simulink model "GD32__HOST"  (R2024a)
settings: Solver=FixedStepDiscrete  StartTime=0.0  StopTime=inf  FixedStep=0.1  RelTol=1e-3
libraries: instrumentseriallib x3
settings Model: Creator=33595  LastModifiedBy=ZJH
settings SolverCC: AlgebraicLoopSolver=TrustRegion
settings DataIOCC: ReturnWorkspaceOutputs=off
settings DebuggingCC: UnconnectedInputMsg=warning  UnconnectedOutputMsg=warning  UnconnectedLineMsg=warning
settings ModelReferenceCC: EnableRefExpFcnMdlSchedulingChecks=on
settings SFSimCC: CustomCodeUndefinedFunction=UseInterfaceOnly
settings RTWCC: GPUComputeCapability=3.5  DLArmComputeVersion=19.05

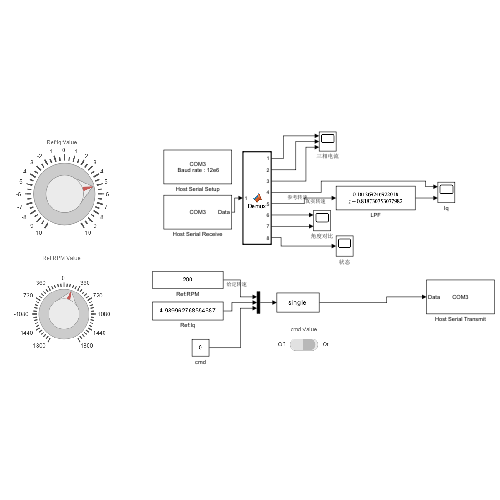
[thumbnail: Simulink's stored preview of the top-level diagram]
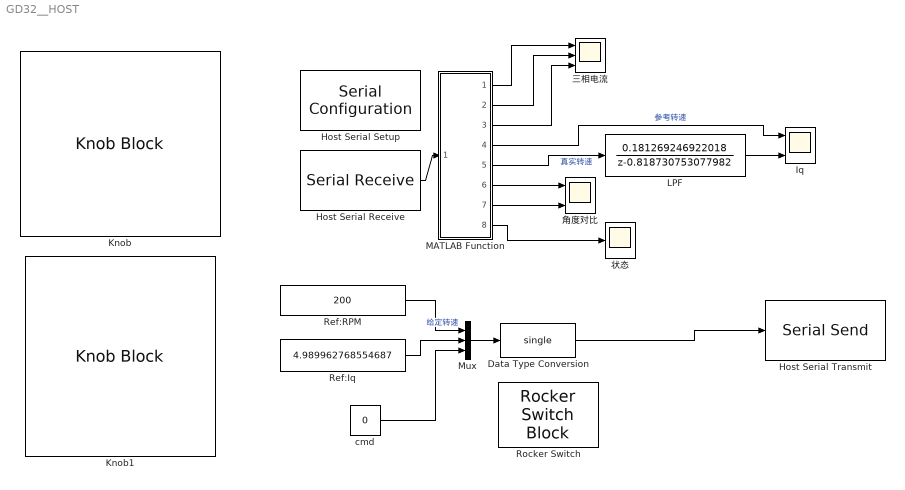
== system GD32__HOST ==
  Data Type Conversion : DataTypeConversion  OutDataTypeStr=single  SaturateOnIntegerOverflow=off  RndMeth=Floor
  Host Serial Receive : instrumentseriallib/Serial Receive  PortSel=COM3  Port=COM3  ComPort=COM3  DataType=single  SaveDataType=uint8  ToggleHeader=off  Header='PMSM'  ToggleDataSize=on  DataSize=[1000 8]  ToggleTerminator=off  Terminator=Custom terminator  CustomTerminator='ATJC'  InputFormat=Row major  EnableBlockingMode=on  ActionDataUnavailable=Output custom value  ActionWhenDataUnavailable=Output custom value  CustomValue=0  SampleTime=0.1  SimulateUsing=Interpreted execution  BlockInModel=on  aMode=5
      settings: LibrarySourceBlock=mcbhostblockslib/Host Serial Receive
  Host Serial Setup : instrumentseriallib/Serial Configuration  Priority=-99  PortSel=COM3  Port=COM3  ComPort=COM3  BaudRate=12e6  DataBits=8  Parity=none  StopBits=1  ByteOrder=little-endian  FlowControl=none  Timeout=1.0  SimulateUsing=Interpreted execution  BlockInModel=on  aMode=5
      settings: LibrarySourceBlock=mcbhostblockslib/Host Serial Setup
  Host Serial Transmit : instrumentseriallib/Serial Send  PortSel=COM3  Port=COM3  ComPort=COM3  Header='ATJC'  Terminator=Custom terminator  CustomTerminator='PMSM'  EnableBlockingMode=off  SimulateUsing=Interpreted execution  BlockInModel=on  aMode=5
      settings: LibrarySourceBlock=mcbhostblockslib/Host Serial Transmit
  Iq : Scope  NumInputPorts=2
  Knob : KnobBlock  ScaleMin=-10  ScaleMax=10
  Knob1 : KnobBlock  ScaleMin=-1800  ScaleMax=1800
  LPF : DiscreteTransferFcn  Numerator=[0.181269246922018]  Denominator=[1 -0.818730753077982]
  MATLAB Function : MATLAB Function  TreatAsAtomicUnit=on
  Mux : Mux  Inputs=3
  Ref:Iq : Constant  Value=4.989962768554687
  Ref:RPM : Constant  Value=200
  Rocker Switch : RockerSwitchBlock
      settings: Values={{'Off', 'On'}, [0 1]}
  cmd : Constant  Value=0
  三相电流 : Scope  NumInputPorts=3
  状态 : Scope
  角度对比 : Scope  NumInputPorts=2
  wires:
  Host Serial Receive/1 -> MATLAB Function/1(Input)
  Ref:RPM/1 -> Mux/1  "给定转速"
  Ref:Iq/1 -> Mux/2
  cmd/1 -> Mux/3
  Data Type Conversion/1 -> Host Serial Transmit/1
  Mux/1 -> Data Type Conversion/1
  MATLAB Function/1(Output1) -> 三相电流/1
  MATLAB Function/2(Output2) -> 三相电流/2
  MATLAB Function/3(Output3) -> 三相电流/3
  MATLAB Function/4(Output4) -> Iq/1  "参考转速"
  MATLAB Function/5(Output5) -> LPF/1  "真实转速"
  MATLAB Function/6(Output6) -> 角度对比/1
  MATLAB Function/7(Output7) -> 角度对比/2
  MATLAB Function/8(Output8) -> 状态/1
  LPF/1 -> Iq/2

== matlab function GD32__HOST/MATLAB Function ==
  data: Input input; Output1 output; Output2 output; Output3 output; Output4 output; Output5 output; Output6 output; Output7 output; Output8 output
function [Output1,Output2,Output3,Output4,Output5,Output6,Output7,Output8]  = Demux(Input)

Output1 = Input(:, 1);
Output2 = Input(:, 2);
Output3 = Input(:, 3);
Output4 = Input(:, 4);
Output5 = Input(:, 5);
Output6 = Input(:, 6);
Output7 = Input(:, 7);
Output8 = Input(:, 8);
end
